simulink model "shower_system_control"  (R2026b)
settings: Solver=ode4  StopTime=60  FixedStep=0.5
undefined symbols (not defined in the file or in its folder): DiscIntNeverNeededParam
settings Model: LastModifiedBy=Ruben
settings DataIOCC: ReturnWorkspaceOutputs=off

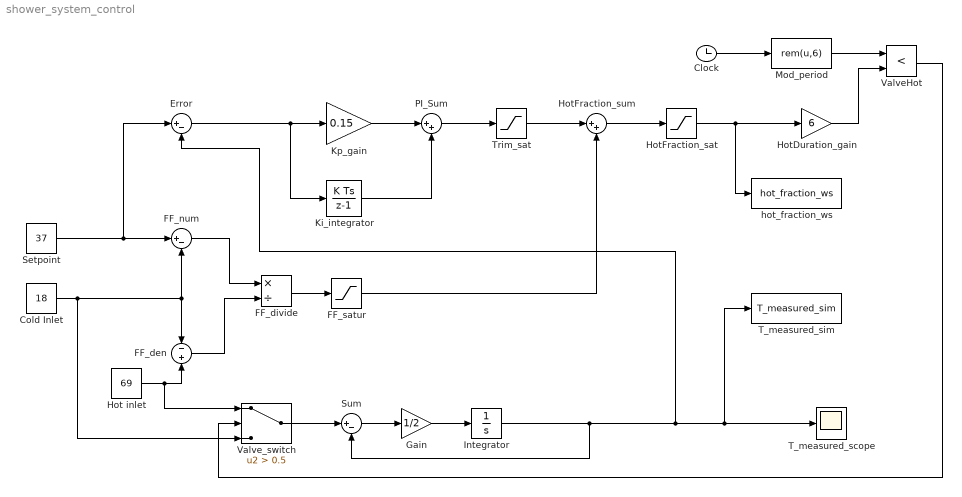
== system shower_system_control ==
  Clock : Clock
  Cold Inlet : Constant  Value=18
  Error : Sum  Inputs=|+-
  FF_den : Sum  Inputs=-+
  FF_divide : Product  Inputs=*/
  FF_num : Sum  Inputs=|+-
  FF_satur : Saturate  UpperLimit=1  LowerLimit=0
  Gain : Gain  Gain=1/2
  Hot inlet : Constant  Value=69
  HotDuration_gain : Gain  Gain=6
  HotFraction_sat : Saturate  UpperLimit=1  LowerLimit=0
  HotFraction_sum : Sum  Inputs=|++
  Integrator : Integrator  InitialCondition=18
  Ki_integrator : DiscreteIntegrator  gainval=0.015  SampleTime=0.5  LimitOutput=on  UpperSaturationLimit=1  LowerSaturationLimit=-1  ICPrevOutput=DiscIntNeverNeededParam  ICPrevScaledInput=DiscIntNeverNeededParam
  Kp_gain : Gain  Gain=0.15
  Mod_period : Fcn  Expr=rem(u,6)
  PI_Sum : Sum  Inputs=|++
  Setpoint : Constant  Value=37
  Sum : Sum  Inputs=|+-
  T_measured_scope : Scope
      settings: ActiveDisplayYMinimum=15.054455429328597  ActiveDisplayYMaximum=44.509901136042636
  T_measured_sim : ToWorkspace  VariableName=T_measured_sim  SaveFormat=Structure With Time  SampleTime=-1
  Trim_sat : Saturate  UpperLimit=1  LowerLimit=-1
  ValveHot : RelationalOperator  Operator=<  OutDataTypeStr=boolean  RndMeth=Simplest  InputSameDT=off
  Valve_switch : Switch  Criteria=u2 > Threshold  Threshold=0.5  SaturateOnIntegerOverflow=off  InputSameDT=off
  hot_fraction_ws : ToWorkspace  VariableName=hot_fraction_ws  SaveFormat=Structure With Time  SampleTime=-1
  wires:
  Setpoint/1 -> Error/1, FF_num/1
  Cold Inlet/1 -> Valve_switch/3, FF_den/1, FF_num/2
  Hot inlet/1 -> Valve_switch/1, FF_den/2
  FF_num/1 -> FF_divide/1
  FF_den/1 -> FF_divide/2
  FF_divide/1 -> FF_satur/1
  Error/1 -> Ki_integrator/1, Kp_gain/1
  PI_Sum/1 -> Trim_sat/1
  FF_satur/1 -> HotFraction_sum/2
  HotFraction_sum/1 -> HotFraction_sat/1
  Trim_sat/1 -> HotFraction_sum/1
  Kp_gain/1 -> PI_Sum/1
  Ki_integrator/1 -> PI_Sum/2
  HotFraction_sat/1 -> hot_fraction_ws/1, HotDuration_gain/1
  Clock/1 -> Mod_period/1
  Mod_period/1 -> ValveHot/1
  HotDuration_gain/1 -> ValveHot/2
  Valve_switch/1 -> Sum/1
  Integrator/1 -> Sum/2, Error/2, T_measured_scope/1, T_measured_sim/1
  ValveHot/1 -> Valve_switch/2
  Sum/1 -> Gain/1
  Gain/1 -> Integrator/1
